simulink model "rfsoc4x2_ospfb_128"  (R2021a)
settings: Solver=VariableStepAuto  StartTime=0.0  StopTime=2048  RelTol=1e-3
undefined symbols (not defined in the file): pfb_coeff_gen_calc
libraries: xbsIndex_r4 x37092, casper_library_delays x737, casper_library_misc x68, xps_library x1
(part 128 of 339)

== system rfsoc4x2_ospfb_128/pfb_fir_real9/pol1_in1_tap27 ==
  din : Inport
  sync : Inport  Port=2
  coeff : Inport  Port=3
  addr_in : Inport  Port=4
  pot_en_in : Inport  Port=5
  Constant59 : xbsIndex_r4/Constant  const=0  gui_display_data_type=Fixed-point  arith_type=Unsigned  n_bits=16  bin_pt=0  preci_type=Single  exp_width=8  frac_width=24  explicit_period=off  period=1  equ=P=C  opselect=C  inp2=PCIN>>17  opr=+  inp1=P  carry=CIN  dbl_ovrd=off  block_type=constant
  Constant60 : xbsIndex_r4/Constant  const=0  gui_display_data_type=Boolean  arith_type=Boolean  n_bits=144  bin_pt=0  preci_type=Single  exp_width=8  frac_width=24  explicit_period=off  period=1  equ=P=C  opselect=C  inp2=PCIN>>17  opr=+  inp1=P  carry=CIN  dbl_ovrd=off  block_type=constant
  Delay : xbsIndex_r4/Delay  rst=off  infoeditControl=Selection of Reset will increase slice count due to use of real FFs and instead of SRLs  en=off  latency=1  reg_retiming=off  dbl_ovrd=off  block_type=delay
  Delay1 : xbsIndex_r4/Delay  rst=off  infoeditControl=Selection of Reset will increase slice count due to use of real FFs and instead of SRLs  en=off  latency=1  reg_retiming=off  dbl_ovrd=off  block_type=delay
  Dual Port RAM13 : xbsIndex_r4/Dual Port RAM  depth=(2^8) / (2^4)  initVector=0  distributed_mem=Block RAM  init_a=0  init_b=0  rst_a=off  rst_b=off  en_a=off  en_b=off  latency=1  write_mode_A=Read After Write  write_mode_B=Read Before Write  optimize=Area  dbl_ovrd=off  simulation_type=fast_sim  block_type=dpram
  Mult : xbsIndex_r4/Mult  precision=Full  arith_type="Signed  (2's comp)"  n_bits=8  bin_pt=2  quantization=Truncate  overflow=Wrap  en=off  latency=0  use_behavioral_HDL=on  opt=Speed  use_embedded=off  optimum_pipeline=off  pipeline=on  dbl_ovrd=off  use_rpm=on  placement_style=Rectangular shape  block_type=mult
      settings: xl_area=[0, 0, 0, 0, 0, 0, 0]  block_version=9.1.01
  Reinterpret : xbsIndex_r4/Reinterpret  force_arith_type=on  arith_type="Signed  (2's comp)"  force_bin_pt=on  bin_pt=coeff_frac_width  block_type=reinterpret
      settings: infoedit="Changes signal type without altering the binary representation.   You can changed the signal between signed and unsigned, and relocate the binary point.<P><P>Hardware notes: In hardware this block costs nothing.<P><P>Example:  Suppose the input is 6 bits wide, signed, with 2 fractional bits, and the output is forced to unsigned with 0 fractional bits.  Then an input of -2.0 (1110.00 in binary 2's complement) becomes an output of 56 (111000 in binary)."  block_version=9.1.01
  Reinterpret1 : xbsIndex_r4/Reinterpret  force_arith_type=on  arith_type="Signed  (2's comp)"  force_bin_pt=on  bin_pt=data_width - 1  block_type=reinterpret
      settings: infoedit="Changes signal type without altering the binary representation.   You can changed the signal between signed and unsigned, and relocate the binary point.<P><P>Hardware notes: In hardware this block costs nothing.<P><P>Example:  Suppose the input is 6 bits wide, signed, with 2 fractional bits, and the output is forced to unsigned with 0 fractional bits.  Then an input of -2.0 (1110.00 in binary 2's complement) becomes an output of 56 (111000 in binary)."  block_version=9.1.01
  Slice : xbsIndex_r4/Slice  nbits=coeff_width  boolean_output=off  mode=Lower Bit Location + Width  bit1=0  base1=MSB of Input  bit0=0  base0=LSB of Input  dbl_ovrd=off  block_type=slice
      settings: infoedit="Extracts a given range of bits from each input sample and presents it at the output.  The output type is ordinarily unsigned with binary point at zero, but can be Boolean when the slice is one bit wide.<P><P>Hardware notes: In hardware this block costs nothing."  block_version=9.1.01
  Slice1 : xbsIndex_r4/Slice  nbits=0  boolean_output=off  mode=Two Bit Locations  bit1=0  base1=MSB of Input  bit0=coeff_width  base0=LSB of Input  dbl_ovrd=off  block_type=slice
      settings: infoedit="Extracts a given range of bits from each input sample and presents it at the output.  The output type is ordinarily unsigned with binary point at zero, but can be Boolean when the slice is one bit wide.<P><P>Hardware notes: In hardware this block costs nothing."  block_version=9.1.01
  Terminator13 : Terminator
  delay_bram : Subsystem  Commented=on  AncestorBlock=casper_library_delays/delay_bram  mask(delay_bram){DelayLen=delay, bram_latency=bram_latency, use_dsp48=off, async=off}
      mask prompts: DelayLen "Delay By:"; bram_latency "BRAM Latency"; use_dsp48 "Use DSP48"; async "asynchronous operation"
      mask help: A delay block that uses BRAM for its storage.
      mask init:
      | delay_bram_init(gcb, ...
      |     'DelayLen', DelayLen, ...
      |     'bram_latency', bram_latency, ...
      |     'use_dsp48', use_dsp48, ...
      |     'async', async);
      mask Help: eval('xlWeb(''http://casper.berkeley.edu/wiki/Delay_bram'')')
  sync_delay : casper_library_delays/sync_delay  DelayLen=delay
      settings: SourceProductName=CASPER DSP Blockset
  dout : Outport  VectorParamsAs1DForOutWhenUnconnected=off
  sync_out : Outport  Port=2  VectorParamsAs1DForOutWhenUnconnected=off
  coeff_out : Outport  Port=3  VectorParamsAs1DForOutWhenUnconnected=off
  taps_out : Outport  Port=4  VectorParamsAs1DForOutWhenUnconnected=off
  add_out : Outport  Port=5  VectorParamsAs1DForOutWhenUnconnected=off
  pot_en_out : Outport  Port=6  VectorParamsAs1DForOutWhenUnconnected=off
  wires:
  addr_in/1 -> Dual Port RAM13/4, Dual Port RAM13/1, Delay/1
  pot_en_in/1 -> Delay1/1, Dual Port RAM13/3
  Constant59/1 -> Dual Port RAM13/5
  Constant60/1 -> Dual Port RAM13/6
  Dual Port RAM13/1 -> Terminator13/1
  din/1 -> Dual Port RAM13/2, Reinterpret1/1
  Delay/1 -> add_out/1
  Dual Port RAM13/2 -> dout/1
  Delay1/1 -> pot_en_out/1
  Reinterpret1/1 -> Mult/1
  Reinterpret/1 -> Mult/2
  Slice/1 -> Reinterpret/1
  Slice1/1 -> coeff_out/1
  coeff/1 -> Slice1/1, Slice/1
  sync_delay/1 -> sync_out/1
  sync/1 -> sync_delay/1
  Mult/1 -> taps_out/1

== system rfsoc4x2_ospfb_128/pfb_fir_real9/pol1_in1_tap28 ==
  note: 11 data in
  note: 12 data out
  din : Inport
  sync : Inport  Port=2
  coeff : Inport  Port=3
  addr_in : Inport  Port=4
  pot_en_in : Inport  Port=5
  Constant59 : xbsIndex_r4/Constant  const=0  gui_display_data_type=Fixed-point  arith_type=Unsigned  n_bits=16  bin_pt=0  preci_type=Single  exp_width=8  frac_width=24  explicit_period=off  period=1  equ=P=C  opselect=C  inp2=PCIN>>17  opr=+  inp1=P  carry=CIN  dbl_ovrd=off  block_type=constant
  Constant60 : xbsIndex_r4/Constant  const=0  gui_display_data_type=Boolean  arith_type=Boolean  n_bits=144  bin_pt=0  preci_type=Single  exp_width=8  frac_width=24  explicit_period=off  period=1  equ=P=C  opselect=C  inp2=PCIN>>17  opr=+  inp1=P  carry=CIN  dbl_ovrd=off  block_type=constant
  Dual Port RAM13 : xbsIndex_r4/Dual Port RAM  depth=(2^8) / (2^4)  initVector=0  distributed_mem=Block RAM  init_a=0  init_b=0  rst_a=off  rst_b=off  en_a=off  en_b=off  latency=1  write_mode_A=Read After Write  write_mode_B=Read Before Write  optimize=Area  dbl_ovrd=off  simulation_type=fast_sim  block_type=dpram
  Mult : xbsIndex_r4/Mult  precision=Full  arith_type="Signed  (2's comp)"  n_bits=8  bin_pt=2  quantization=Truncate  overflow=Wrap  en=off  latency=0  use_behavioral_HDL=on  opt=Speed  use_embedded=off  optimum_pipeline=off  pipeline=on  dbl_ovrd=off  use_rpm=on  placement_style=Rectangular shape  block_type=mult
      settings: xl_area=[0, 0, 0, 0, 0, 0, 0]  block_version=9.1.01
  Reinterpret : xbsIndex_r4/Reinterpret  force_arith_type=on  arith_type="Signed  (2's comp)"  force_bin_pt=on  bin_pt=coeff_frac_width  block_type=reinterpret
      settings: infoedit="Changes signal type without altering the binary representation.   You can changed the signal between signed and unsigned, and relocate the binary point.<P><P>Hardware notes: In hardware this block costs nothing.<P><P>Example:  Suppose the input is 6 bits wide, signed, with 2 fractional bits, and the output is forced to unsigned with 0 fractional bits.  Then an input of -2.0 (1110.00 in binary 2's complement) becomes an output of 56 (111000 in binary)."  block_version=9.1.01
  Reinterpret1 : xbsIndex_r4/Reinterpret  force_arith_type=on  arith_type="Signed  (2's comp)"  force_bin_pt=on  bin_pt=data_width - 1  block_type=reinterpret
      settings: infoedit="Changes signal type without altering the binary representation.   You can changed the signal between signed and unsigned, and relocate the binary point.<P><P>Hardware notes: In hardware this block costs nothing.<P><P>Example:  Suppose the input is 6 bits wide, signed, with 2 fractional bits, and the output is forced to unsigned with 0 fractional bits.  Then an input of -2.0 (1110.00 in binary 2's complement) becomes an output of 56 (111000 in binary)."  block_version=9.1.01
  Slice : xbsIndex_r4/Slice  nbits=coeff_width  boolean_output=off  mode=Lower Bit Location + Width  bit1=0  base1=MSB of Input  bit0=0  base0=LSB of Input  dbl_ovrd=off  block_type=slice
      settings: infoedit="Extracts a given range of bits from each input sample and presents it at the output.  The output type is ordinarily unsigned with binary point at zero, but can be Boolean when the slice is one bit wide.<P><P>Hardware notes: In hardware this block costs nothing."  block_version=9.1.01
  Slice1 : xbsIndex_r4/Slice  nbits=0  boolean_output=off  mode=Two Bit Locations  bit1=0  base1=MSB of Input  bit0=coeff_width  base0=LSB of Input  dbl_ovrd=off  block_type=slice
      settings: infoedit="Extracts a given range of bits from each input sample and presents it at the output.  The output type is ordinarily unsigned with binary point at zero, but can be Boolean when the slice is one bit wide.<P><P>Hardware notes: In hardware this block costs nothing."  block_version=9.1.01
  Terminator13 : Terminator
  delay_bram : Subsystem  Commented=on  AncestorBlock=casper_library_delays/delay_bram  mask(delay_bram){DelayLen=delay, bram_latency=bram_latency, use_dsp48=off, async=off}
      mask prompts: DelayLen "Delay By:"; bram_latency "BRAM Latency"; use_dsp48 "Use DSP48"; async "asynchronous operation"
      mask help: A delay block that uses BRAM for its storage.
      mask init:
      | delay_bram_init(gcb, ...
      |     'DelayLen', DelayLen, ...
      |     'bram_latency', bram_latency, ...
      |     'use_dsp48', use_dsp48, ...
      |     'async', async);
      mask Help: eval('xlWeb(''http://casper.berkeley.edu/wiki/Delay_bram'')')
  sync_delay : casper_library_delays/sync_delay  DelayLen=delay
      settings: SourceProductName=CASPER DSP Blockset
  dout : Outport  VectorParamsAs1DForOutWhenUnconnected=off
  sync_out : Outport  Port=2  VectorParamsAs1DForOutWhenUnconnected=off
  coeff_out : Outport  Port=3  VectorParamsAs1DForOutWhenUnconnected=off
  taps_out : Outport  Port=4  VectorParamsAs1DForOutWhenUnconnected=off
  wires:
  Dual Port RAM13/1 -> Terminator13/1
  Dual Port RAM13/2 -> dout/1
  Constant59/1 -> Dual Port RAM13/5
  Constant60/1 -> Dual Port RAM13/6
  din/1 -> Dual Port RAM13/2, Reinterpret1/1
  addr_in/1 -> Dual Port RAM13/1, Dual Port RAM13/4
  pot_en_in/1 -> Dual Port RAM13/3
  Reinterpret1/1 -> Mult/1
  Reinterpret/1 -> Mult/2
  Slice/1 -> Reinterpret/1
  Slice1/1 -> coeff_out/1
  coeff/1 -> Slice1/1, Slice/1
  sync_delay/1 -> sync_out/1
  sync/1 -> sync_delay/1
  Mult/1 -> taps_out/1

== system rfsoc4x2_ospfb_128/pfb_fir_real9/pol1_in1_tap29 ==
  din : Inport
  sync : Inport  Port=2
  coeff : Inport  Port=3
  addr_in : Inport  Port=4
  pot_en_in : Inport  Port=5
  Constant59 : xbsIndex_r4/Constant  const=0  gui_display_data_type=Fixed-point  arith_type=Unsigned  n_bits=16  bin_pt=0  preci_type=Single  exp_width=8  frac_width=24  explicit_period=off  period=1  equ=P=C  opselect=C  inp2=PCIN>>17  opr=+  inp1=P  carry=CIN  dbl_ovrd=off  block_type=constant
  Constant60 : xbsIndex_r4/Constant  const=0  gui_display_data_type=Boolean  arith_type=Boolean  n_bits=144  bin_pt=0  preci_type=Single  exp_width=8  frac_width=24  explicit_period=off  period=1  equ=P=C  opselect=C  inp2=PCIN>>17  opr=+  inp1=P  carry=CIN  dbl_ovrd=off  block_type=constant
  Delay : xbsIndex_r4/Delay  rst=off  infoeditControl=Selection of Reset will increase slice count due to use of real FFs and instead of SRLs  en=off  latency=1  reg_retiming=off  dbl_ovrd=off  block_type=delay
  Delay1 : xbsIndex_r4/Delay  rst=off  infoeditControl=Selection of Reset will increase slice count due to use of real FFs and instead of SRLs  en=off  latency=1  reg_retiming=off  dbl_ovrd=off  block_type=delay
  Dual Port RAM13 : xbsIndex_r4/Dual Port RAM  depth=(2^8) / (2^4)  initVector=0  distributed_mem=Block RAM  init_a=0  init_b=0  rst_a=off  rst_b=off  en_a=off  en_b=off  latency=1  write_mode_A=Read After Write  write_mode_B=Read Before Write  optimize=Area  dbl_ovrd=off  simulation_type=fast_sim  block_type=dpram
  Mult : xbsIndex_r4/Mult  precision=Full  arith_type="Signed  (2's comp)"  n_bits=8  bin_pt=2  quantization=Truncate  overflow=Wrap  en=off  latency=0  use_behavioral_HDL=on  opt=Speed  use_embedded=off  optimum_pipeline=off  pipeline=on  dbl_ovrd=off  use_rpm=on  placement_style=Rectangular shape  block_type=mult
      settings: xl_area=[0, 0, 0, 0, 0, 0, 0]  block_version=9.1.01
  Reinterpret : xbsIndex_r4/Reinterpret  force_arith_type=on  arith_type="Signed  (2's comp)"  force_bin_pt=on  bin_pt=coeff_frac_width  block_type=reinterpret
      settings: infoedit="Changes signal type without altering the binary representation.   You can changed the signal between signed and unsigned, and relocate the binary point.<P><P>Hardware notes: In hardware this block costs nothing.<P><P>Example:  Suppose the input is 6 bits wide, signed, with 2 fractional bits, and the output is forced to unsigned with 0 fractional bits.  Then an input of -2.0 (1110.00 in binary 2's complement) becomes an output of 56 (111000 in binary)."  block_version=9.1.01
  Reinterpret1 : xbsIndex_r4/Reinterpret  force_arith_type=on  arith_type="Signed  (2's comp)"  force_bin_pt=on  bin_pt=data_width - 1  block_type=reinterpret
      settings: infoedit="Changes signal type without altering the binary representation.   You can changed the signal between signed and unsigned, and relocate the binary point.<P><P>Hardware notes: In hardware this block costs nothing.<P><P>Example:  Suppose the input is 6 bits wide, signed, with 2 fractional bits, and the output is forced to unsigned with 0 fractional bits.  Then an input of -2.0 (1110.00 in binary 2's complement) becomes an output of 56 (111000 in binary)."  block_version=9.1.01
  Slice : xbsIndex_r4/Slice  nbits=coeff_width  boolean_output=off  mode=Lower Bit Location + Width  bit1=0  base1=MSB of Input  bit0=0  base0=LSB of Input  dbl_ovrd=off  block_type=slice
      settings: infoedit="Extracts a given range of bits from each input sample and presents it at the output.  The output type is ordinarily unsigned with binary point at zero, but can be Boolean when the slice is one bit wide.<P><P>Hardware notes: In hardware this block costs nothing."  block_version=9.1.01
  Slice1 : xbsIndex_r4/Slice  nbits=0  boolean_output=off  mode=Two Bit Locations  bit1=0  base1=MSB of Input  bit0=coeff_width  base0=LSB of Input  dbl_ovrd=off  block_type=slice
      settings: infoedit="Extracts a given range of bits from each input sample and presents it at the output.  The output type is ordinarily unsigned with binary point at zero, but can be Boolean when the slice is one bit wide.<P><P>Hardware notes: In hardware this block costs nothing."  block_version=9.1.01
  Terminator13 : Terminator
  delay_bram : Subsystem  Commented=on  AncestorBlock=casper_library_delays/delay_bram  mask(delay_bram){DelayLen=delay, bram_latency=bram_latency, use_dsp48=off, async=off}
      mask prompts: DelayLen "Delay By:"; bram_latency "BRAM Latency"; use_dsp48 "Use DSP48"; async "asynchronous operation"
      mask help: A delay block that uses BRAM for its storage.
      mask init:
      | delay_bram_init(gcb, ...
      |     'DelayLen', DelayLen, ...
      |     'bram_latency', bram_latency, ...
      |     'use_dsp48', use_dsp48, ...
      |     'async', async);
      mask Help: eval('xlWeb(''http://casper.berkeley.edu/wiki/Delay_bram'')')
  sync_delay : casper_library_delays/sync_delay  DelayLen=delay
      settings: SourceProductName=CASPER DSP Blockset
  dout : Outport  VectorParamsAs1DForOutWhenUnconnected=off
  sync_out : Outport  Port=2  VectorParamsAs1DForOutWhenUnconnected=off
  coeff_out : Outport  Port=3  VectorParamsAs1DForOutWhenUnconnected=off
  taps_out : Outport  Port=4  VectorParamsAs1DForOutWhenUnconnected=off
  add_out : Outport  Port=5  VectorParamsAs1DForOutWhenUnconnected=off
  pot_en_out : Outport  Port=6  VectorParamsAs1DForOutWhenUnconnected=off
  wires:
  pot_en_in/1 -> Delay1/1, Dual Port RAM13/3
  Constant59/1 -> Dual Port RAM13/5
  Dual Port RAM13/1 -> Terminator13/1
  Dual Port RAM13/2 -> dout/1
  addr_in/1 -> Dual Port RAM13/4, Dual Port RAM13/1, Delay/1
  Delay/1 -> add_out/1
  Delay1/1 -> pot_en_out/1
  din/1 -> Dual Port RAM13/2, Reinterpret1/1
  Constant60/1 -> Dual Port RAM13/6
  Reinterpret1/1 -> Mult/1
  Reinterpret/1 -> Mult/2
  Slice/1 -> Reinterpret/1
  Slice1/1 -> coeff_out/1
  coeff/1 -> Slice1/1, Slice/1
  sync_delay/1 -> sync_out/1
  sync/1 -> sync_delay/1
  Mult/1 -> taps_out/1

== system rfsoc4x2_ospfb_128/pfb_fir_real9/pol1_in1_tap3 ==
  din : Inport
  sync : Inport  Port=2
  coeff : Inport  Port=3
  addr_in : Inport  Port=4
  pot_en_in : Inport  Port=5
  Constant59 : xbsIndex_r4/Constant  const=0  gui_display_data_type=Fixed-point  arith_type=Unsigned  n_bits=16  bin_pt=0  preci_type=Single  exp_width=8  frac_width=24  explicit_period=off  period=1  equ=P=C  opselect=C  inp2=PCIN>>17  opr=+  inp1=P  carry=CIN  dbl_ovrd=off  block_type=constant
  Constant60 : xbsIndex_r4/Constant  const=0  gui_display_data_type=Boolean  arith_type=Boolean  n_bits=144  bin_pt=0  preci_type=Single  exp_width=8  frac_width=24  explicit_period=off  period=1  equ=P=C  opselect=C  inp2=PCIN>>17  opr=+  inp1=P  carry=CIN  dbl_ovrd=off  block_type=constant
  Delay : xbsIndex_r4/Delay  rst=off  infoeditControl=Selection of Reset will increase slice count due to use of real FFs and instead of SRLs  en=off  latency=1  reg_retiming=off  dbl_ovrd=off  block_type=delay
  Delay1 : xbsIndex_r4/Delay  rst=off  infoeditControl=Selection of Reset will increase slice count due to use of real FFs and instead of SRLs  en=off  latency=1  reg_retiming=off  dbl_ovrd=off  block_type=delay
  Dual Port RAM13 : xbsIndex_r4/Dual Port RAM  depth=(2^8) / (2^4)  initVector=0  distributed_mem=Block RAM  init_a=0  init_b=0  rst_a=off  rst_b=off  en_a=off  en_b=off  latency=1  write_mode_A=Read After Write  write_mode_B=Read Before Write  optimize=Area  dbl_ovrd=off  simulation_type=fast_sim  block_type=dpram
  Mult : xbsIndex_r4/Mult  precision=Full  arith_type="Signed  (2's comp)"  n_bits=8  bin_pt=2  quantization=Truncate  overflow=Wrap  en=off  latency=0  use_behavioral_HDL=on  opt=Speed  use_embedded=off  optimum_pipeline=off  pipeline=on  dbl_ovrd=off  use_rpm=on  placement_style=Rectangular shape  block_type=mult
      settings: xl_area=[0, 0, 0, 0, 0, 0, 0]  block_version=9.1.01
  Reinterpret : xbsIndex_r4/Reinterpret  force_arith_type=on  arith_type="Signed  (2's comp)"  force_bin_pt=on  bin_pt=coeff_frac_width  block_type=reinterpret
      settings: infoedit="Changes signal type without altering the binary representation.   You can changed the signal between signed and unsigned, and relocate the binary point.<P><P>Hardware notes: In hardware this block costs nothing.<P><P>Example:  Suppose the input is 6 bits wide, signed, with 2 fractional bits, and the output is forced to unsigned with 0 fractional bits.  Then an input of -2.0 (1110.00 in binary 2's complement) becomes an output of 56 (111000 in binary)."  block_version=9.1.01
  Reinterpret1 : xbsIndex_r4/Reinterpret  force_arith_type=on  arith_type="Signed  (2's comp)"  force_bin_pt=on  bin_pt=data_width - 1  block_type=reinterpret
      settings: infoedit="Changes signal type without altering the binary representation.   You can changed the signal between signed and unsigned, and relocate the binary point.<P><P>Hardware notes: In hardware this block costs nothing.<P><P>Example:  Suppose the input is 6 bits wide, signed, with 2 fractional bits, and the output is forced to unsigned with 0 fractional bits.  Then an input of -2.0 (1110.00 in binary 2's complement) becomes an output of 56 (111000 in binary)."  block_version=9.1.01
  Slice : xbsIndex_r4/Slice  nbits=coeff_width  boolean_output=off  mode=Lower Bit Location + Width  bit1=0  base1=MSB of Input  bit0=0  base0=LSB of Input  dbl_ovrd=off  block_type=slice
      settings: infoedit="Extracts a given range of bits from each input sample and presents it at the output.  The output type is ordinarily unsigned with binary point at zero, but can be Boolean when the slice is one bit wide.<P><P>Hardware notes: In hardware this block costs nothing."  block_version=9.1.01
  Slice1 : xbsIndex_r4/Slice  nbits=0  boolean_output=off  mode=Two Bit Locations  bit1=0  base1=MSB of Input  bit0=coeff_width  base0=LSB of Input  dbl_ovrd=off  block_type=slice
      settings: infoedit="Extracts a given range of bits from each input sample and presents it at the output.  The output type is ordinarily unsigned with binary point at zero, but can be Boolean when the slice is one bit wide.<P><P>Hardware notes: In hardware this block costs nothing."  block_version=9.1.01
  Terminator13 : Terminator
  delay_bram : Subsystem  Commented=on  AncestorBlock=casper_library_delays/delay_bram  mask(delay_bram){DelayLen=delay, bram_latency=bram_latency, use_dsp48=off, async=off}
      mask prompts: DelayLen "Delay By:"; bram_latency "BRAM Latency"; use_dsp48 "Use DSP48"; async "asynchronous operation"
      mask help: A delay block that uses BRAM for its storage.
      mask init:
      | delay_bram_init(gcb, ...
      |     'DelayLen', DelayLen, ...
      |     'bram_latency', bram_latency, ...
      |     'use_dsp48', use_dsp48, ...
      |     'async', async);
      mask Help: eval('xlWeb(''http://casper.berkeley.edu/wiki/Delay_bram'')')
  sync_delay : casper_library_delays/sync_delay  DelayLen=delay
      settings: SourceProductName=CASPER DSP Blockset
  dout : Outport  VectorParamsAs1DForOutWhenUnconnected=off
  sync_out : Outport  Port=2  VectorParamsAs1DForOutWhenUnconnected=off
  coeff_out : Outport  Port=3  VectorParamsAs1DForOutWhenUnconnected=off
  taps_out : Outport  Port=4  VectorParamsAs1DForOutWhenUnconnected=off
  add_out : Outport  Port=5  VectorParamsAs1DForOutWhenUnconnected=off
  pot_en_out : Outport  Port=6  VectorParamsAs1DForOutWhenUnconnected=off
  wires:
  Mult/1 -> taps_out/1
  sync/1 -> sync_delay/1
  sync_delay/1 -> sync_out/1
  coeff/1 -> Slice/1, Slice1/1
  Slice1/1 -> coeff_out/1
  Slice/1 -> Reinterpret/1
  Reinterpret/1 -> Mult/2
  Reinterpret1/1 -> Mult/1
  Constant60/1 -> Dual Port RAM13/6
  din/1 -> Reinterpret1/1, Dual Port RAM13/2
  Delay1/1 -> pot_en_out/1
  Delay/1 -> add_out/1
  addr_in/1 -> Delay/1, Dual Port RAM13/1, Dual Port RAM13/4
  Dual Port RAM13/2 -> dout/1
  Dual Port RAM13/1 -> Terminator13/1
  Constant59/1 -> Dual Port RAM13/5
  pot_en_in/1 -> Dual Port RAM13/3, Delay1/1

== system rfsoc4x2_ospfb_128/pfb_fir_real9/pol1_in1_tap30 ==
  din : Inport
  sync : Inport  Port=2
  coeff : Inport  Port=3
  addr_in : Inport  Port=4
  pot_en_in : Inport  Port=5
  Constant59 : xbsIndex_r4/Constant  const=0  gui_display_data_type=Fixed-point  arith_type=Unsigned  n_bits=16  bin_pt=0  preci_type=Single  exp_width=8  frac_width=24  explicit_period=off  period=1  equ=P=C  opselect=C  inp2=PCIN>>17  opr=+  inp1=P  carry=CIN  dbl_ovrd=off  block_type=constant
  Constant60 : xbsIndex_r4/Constant  const=0  gui_display_data_type=Boolean  arith_type=Boolean  n_bits=144  bin_pt=0  preci_type=Single  exp_width=8  frac_width=24  explicit_period=off  period=1  equ=P=C  opselect=C  inp2=PCIN>>17  opr=+  inp1=P  carry=CIN  dbl_ovrd=off  block_type=constant
  Delay : xbsIndex_r4/Delay  rst=off  infoeditControl=Selection of Reset will increase slice count due to use of real FFs and instead of SRLs  en=off  latency=1  reg_retiming=off  dbl_ovrd=off  block_type=delay
  Delay1 : xbsIndex_r4/Delay  rst=off  infoeditControl=Selection of Reset will increase slice count due to use of real FFs and instead of SRLs  en=off  latency=1  reg_retiming=off  dbl_ovrd=off  block_type=delay
  Dual Port RAM13 : xbsIndex_r4/Dual Port RAM  depth=(2^8) / (2^4)  initVector=0  distributed_mem=Block RAM  init_a=0  init_b=0  rst_a=off  rst_b=off  en_a=off  en_b=off  latency=1  write_mode_A=Read After Write  write_mode_B=Read Before Write  optimize=Area  dbl_ovrd=off  simulation_type=fast_sim  block_type=dpram
  Mult : xbsIndex_r4/Mult  precision=Full  arith_type="Signed  (2's comp)"  n_bits=8  bin_pt=2  quantization=Truncate  overflow=Wrap  en=off  latency=0  use_behavioral_HDL=on  opt=Speed  use_embedded=off  optimum_pipeline=off  pipeline=on  dbl_ovrd=off  use_rpm=on  placement_style=Rectangular shape  block_type=mult
      settings: xl_area=[0, 0, 0, 0, 0, 0, 0]  block_version=9.1.01
  Reinterpret : xbsIndex_r4/Reinterpret  force_arith_type=on  arith_type="Signed  (2's comp)"  force_bin_pt=on  bin_pt=coeff_frac_width  block_type=reinterpret
      settings: infoedit="Changes signal type without altering the binary representation.   You can changed the signal between signed and unsigned, and relocate the binary point.<P><P>Hardware notes: In hardware this block costs nothing.<P><P>Example:  Suppose the input is 6 bits wide, signed, with 2 fractional bits, and the output is forced to unsigned with 0 fractional bits.  Then an input of -2.0 (1110.00 in binary 2's complement) becomes an output of 56 (111000 in binary)."  block_version=9.1.01
  Reinterpret1 : xbsIndex_r4/Reinterpret  force_arith_type=on  arith_type="Signed  (2's comp)"  force_bin_pt=on  bin_pt=data_width - 1  block_type=reinterpret
      settings: infoedit="Changes signal type without altering the binary representation.   You can changed the signal between signed and unsigned, and relocate the binary point.<P><P>Hardware notes: In hardware this block costs nothing.<P><P>Example:  Suppose the input is 6 bits wide, signed, with 2 fractional bits, and the output is forced to unsigned with 0 fractional bits.  Then an input of -2.0 (1110.00 in binary 2's complement) becomes an output of 56 (111000 in binary)."  block_version=9.1.01
  Slice : xbsIndex_r4/Slice  nbits=coeff_width  boolean_output=off  mode=Lower Bit Location + Width  bit1=0  base1=MSB of Input  bit0=0  base0=LSB of Input  dbl_ovrd=off  block_type=slice
      settings: infoedit="Extracts a given range of bits from each input sample and presents it at the output.  The output type is ordinarily unsigned with binary point at zero, but can be Boolean when the slice is one bit wide.<P><P>Hardware notes: In hardware this block costs nothing."  block_version=9.1.01
  Slice1 : xbsIndex_r4/Slice  nbits=0  boolean_output=off  mode=Two Bit Locations  bit1=0  base1=MSB of Input  bit0=coeff_width  base0=LSB of Input  dbl_ovrd=off  block_type=slice
      settings: infoedit="Extracts a given range of bits from each input sample and presents it at the output.  The output type is ordinarily unsigned with binary point at zero, but can be Boolean when the slice is one bit wide.<P><P>Hardware notes: In hardware this block costs nothing."  block_version=9.1.01
  Terminator13 : Terminator
  delay_bram : Subsystem  Commented=on  AncestorBlock=casper_library_delays/delay_bram  mask(delay_bram){DelayLen=delay, bram_latency=bram_latency, use_dsp48=off, async=off}
      mask prompts: DelayLen "Delay By:"; bram_latency "BRAM Latency"; use_dsp48 "Use DSP48"; async "asynchronous operation"
      mask help: A delay block that uses BRAM for its storage.
      mask init:
      | delay_bram_init(gcb, ...
      |     'DelayLen', DelayLen, ...
      |     'bram_latency', bram_latency, ...
      |     'use_dsp48', use_dsp48, ...
      |     'async', async);
      mask Help: eval('xlWeb(''http://casper.berkeley.edu/wiki/Delay_bram'')')
  sync_delay : casper_library_delays/sync_delay  DelayLen=delay
      settings: SourceProductName=CASPER DSP Blockset
  dout : Outport  VectorParamsAs1DForOutWhenUnconnected=off
  sync_out : Outport  Port=2  VectorParamsAs1DForOutWhenUnconnected=off
  coeff_out : Outport  Port=3  VectorParamsAs1DForOutWhenUnconnected=off
  taps_out : Outport  Port=4  VectorParamsAs1DForOutWhenUnconnected=off
  add_out : Outport  Port=5  VectorParamsAs1DForOutWhenUnconnected=off
  pot_en_out : Outport  Port=6  VectorParamsAs1DForOutWhenUnconnected=off
  wires:
  addr_in/1 -> Dual Port RAM13/4, Dual Port RAM13/1, Delay/1
  pot_en_in/1 -> Delay1/1, Dual Port RAM13/3
  Constant59/1 -> Dual Port RAM13/5
  Constant60/1 -> Dual Port RAM13/6
  Dual Port RAM13/1 -> Terminator13/1
  din/1 -> Reinterpret1/1, Dual Port RAM13/2
  Delay/1 -> add_out/1
  Dual Port RAM13/2 -> dout/1
  Delay1/1 -> pot_en_out/1
  Reinterpret1/1 -> Mult/1
  Reinterpret/1 -> Mult/2
  Slice/1 -> Reinterpret/1
  Slice1/1 -> coeff_out/1
  coeff/1 -> Slice1/1, Slice/1
  sync_delay/1 -> sync_out/1
  sync/1 -> sync_delay/1
  Mult/1 -> taps_out/1

== system rfsoc4x2_ospfb_128/pfb_fir_real9/pol1_in1_tap31 ==
  note: 10 data in
  note: 11 data out
  din : Inport
  sync : Inport  Port=2
  coeff : Inport  Port=3
  addr_in : Inport  Port=4
  pot_en_in : Inport  Port=5
  Constant59 : xbsIndex_r4/Constant  const=0  gui_display_data_type=Fixed-point  arith_type=Unsigned  n_bits=16  bin_pt=0  preci_type=Single  exp_width=8  frac_width=24  explicit_period=off  period=1  equ=P=C  opselect=C  inp2=PCIN>>17  opr=+  inp1=P  carry=CIN  dbl_ovrd=off  block_type=constant
  Constant60 : xbsIndex_r4/Constant  const=0  gui_display_data_type=Boolean  arith_type=Boolean  n_bits=144  bin_pt=0  preci_type=Single  exp_width=8  frac_width=24  explicit_period=off  period=1  equ=P=C  opselect=C  inp2=PCIN>>17  opr=+  inp1=P  carry=CIN  dbl_ovrd=off  block_type=constant
  Delay : xbsIndex_r4/Delay  rst=off  infoeditControl=Selection of Reset will increase slice count due to use of real FFs and instead of SRLs  en=off  latency=1  reg_retiming=off  dbl_ovrd=off  block_type=delay
  Delay1 : xbsIndex_r4/Delay  rst=off  infoeditControl=Selection of Reset will increase slice count due to use of real FFs and instead of SRLs  en=off  latency=1  reg_retiming=off  dbl_ovrd=off  block_type=delay
  Dual Port RAM13 : xbsIndex_r4/Dual Port RAM  depth=(2^8) / (2^4)  initVector=0  distributed_mem=Block RAM  init_a=0  init_b=0  rst_a=off  rst_b=off  en_a=off  en_b=off  latency=1  write_mode_A=Read After Write  write_mode_B=Read Before Write  optimize=Area  dbl_ovrd=off  simulation_type=fast_sim  block_type=dpram
  Mult : xbsIndex_r4/Mult  precision=Full  arith_type="Signed  (2's comp)"  n_bits=8  bin_pt=2  quantization=Truncate  overflow=Wrap  en=off  latency=0  use_behavioral_HDL=on  opt=Speed  use_embedded=off  optimum_pipeline=off  pipeline=on  dbl_ovrd=off  use_rpm=on  placement_style=Rectangular shape  block_type=mult
      settings: xl_area=[0, 0, 0, 0, 0, 0, 0]  block_version=9.1.01
  Reinterpret : xbsIndex_r4/Reinterpret  force_arith_type=on  arith_type="Signed  (2's comp)"  force_bin_pt=on  bin_pt=coeff_frac_width  block_type=reinterpret
      settings: infoedit="Changes signal type without altering the binary representation.   You can changed the signal between signed and unsigned, and relocate the binary point.<P><P>Hardware notes: In hardware this block costs nothing.<P><P>Example:  Suppose the input is 6 bits wide, signed, with 2 fractional bits, and the output is forced to unsigned with 0 fractional bits.  Then an input of -2.0 (1110.00 in binary 2's complement) becomes an output of 56 (111000 in binary)."  block_version=9.1.01
  Reinterpret1 : xbsIndex_r4/Reinterpret  force_arith_type=on  arith_type="Signed  (2's comp)"  force_bin_pt=on  bin_pt=data_width - 1  block_type=reinterpret
      settings: infoedit="Changes signal type without altering the binary representation.   You can changed the signal between signed and unsigned, and relocate the binary point.<P><P>Hardware notes: In hardware this block costs nothing.<P><P>Example:  Suppose the input is 6 bits wide, signed, with 2 fractional bits, and the output is forced to unsigned with 0 fractional bits.  Then an input of -2.0 (1110.00 in binary 2's complement) becomes an output of 56 (111000 in binary)."  block_version=9.1.01
  Slice : xbsIndex_r4/Slice  nbits=coeff_width  boolean_output=off  mode=Lower Bit Location + Width  bit1=0  base1=MSB of Input  bit0=0  base0=LSB of Input  dbl_ovrd=off  block_type=slice
      settings: infoedit="Extracts a given range of bits from each input sample and presents it at the output.  The output type is ordinarily unsigned with binary point at zero, but can be Boolean when the slice is one bit wide.<P><P>Hardware notes: In hardware this block costs nothing."  block_version=9.1.01
  Slice1 : xbsIndex_r4/Slice  nbits=0  boolean_output=off  mode=Two Bit Locations  bit1=0  base1=MSB of Input  bit0=coeff_width  base0=LSB of Input  dbl_ovrd=off  block_type=slice
      settings: infoedit="Extracts a given range of bits from each input sample and presents it at the output.  The output type is ordinarily unsigned with binary point at zero, but can be Boolean when the slice is one bit wide.<P><P>Hardware notes: In hardware this block costs nothing."  block_version=9.1.01
  Terminator13 : Terminator
  delay_bram : Subsystem  Commented=on  AncestorBlock=casper_library_delays/delay_bram  mask(delay_bram){DelayLen=delay, bram_latency=bram_latency, use_dsp48=off, async=off}
      mask prompts: DelayLen "Delay By:"; bram_latency "BRAM Latency"; use_dsp48 "Use DSP48"; async "asynchronous operation"
      mask help: A delay block that uses BRAM for its storage.
      mask init:
      | delay_bram_init(gcb, ...
      |     'DelayLen', DelayLen, ...
      |     'bram_latency', bram_latency, ...
      |     'use_dsp48', use_dsp48, ...
      |     'async', async);
      mask Help: eval('xlWeb(''http://casper.berkeley.edu/wiki/Delay_bram'')')
  sync_delay : casper_library_delays/sync_delay  DelayLen=delay
      settings: SourceProductName=CASPER DSP Blockset
  dout : Outport  VectorParamsAs1DForOutWhenUnconnected=off
  sync_out : Outport  Port=2  VectorParamsAs1DForOutWhenUnconnected=off
  coeff_out : Outport  Port=3  VectorParamsAs1DForOutWhenUnconnected=off
  taps_out : Outport  Port=4  VectorParamsAs1DForOutWhenUnconnected=off
  add_out : Outport  Port=5  VectorParamsAs1DForOutWhenUnconnected=off
  pot_en_out : Outport  Port=6  VectorParamsAs1DForOutWhenUnconnected=off
  wires:
  Constant60/1 -> Dual Port RAM13/6
  Delay1/1 -> pot_en_out/1
  Dual Port RAM13/1 -> Terminator13/1
  pot_en_in/1 -> Delay1/1, Dual Port RAM13/3
  Constant59/1 -> Dual Port RAM13/5
  addr_in/1 -> Dual Port RAM13/4, Dual Port RAM13/1, Delay/1
  Dual Port RAM13/2 -> dout/1
  Delay/1 -> add_out/1
  din/1 -> Dual Port RAM13/2, Reinterpret1/1
  Reinterpret1/1 -> Mult/1
  Reinterpret/1 -> Mult/2
  Slice/1 -> Reinterpret/1
  Slice1/1 -> coeff_out/1
  coeff/1 -> Slice1/1, Slice/1
  sync_delay/1 -> sync_out/1
  sync/1 -> sync_delay/1
  Mult/1 -> taps_out/1

== system rfsoc4x2_ospfb_128/pfb_fir_real9/pol1_in1_tap32 ==
  din : Inport
  sync : Inport  Port=2
  coeff : Inport  Port=3
  addr_in : Inport  Port=4
  pot_en_in : Inport  Port=5
  Constant59 : xbsIndex_r4/Constant  const=0  gui_display_data_type=Fixed-point  arith_type=Unsigned  n_bits=16  bin_pt=0  preci_type=Single  exp_width=8  frac_width=24  explicit_period=off  period=1  equ=P=C  opselect=C  inp2=PCIN>>17  opr=+  inp1=P  carry=CIN  dbl_ovrd=off  block_type=constant
  Constant60 : xbsIndex_r4/Constant  const=0  gui_display_data_type=Boolean  arith_type=Boolean  n_bits=144  bin_pt=0  preci_type=Single  exp_width=8  frac_width=24  explicit_period=off  period=1  equ=P=C  opselect=C  inp2=PCIN>>17  opr=+  inp1=P  carry=CIN  dbl_ovrd=off  block_type=constant
  Delay : xbsIndex_r4/Delay  rst=off  infoeditControl=Selection of Reset will increase slice count due to use of real FFs and instead of SRLs  en=off  latency=1  reg_retiming=off  dbl_ovrd=off  block_type=delay
  Delay1 : xbsIndex_r4/Delay  rst=off  infoeditControl=Selection of Reset will increase slice count due to use of real FFs and instead of SRLs  en=off  latency=1  reg_retiming=off  dbl_ovrd=off  block_type=delay
  Dual Port RAM13 : xbsIndex_r4/Dual Port RAM  depth=(2^8) / (2^4)  initVector=0  distributed_mem=Block RAM  init_a=0  init_b=0  rst_a=off  rst_b=off  en_a=off  en_b=off  latency=1  write_mode_A=Read After Write  write_mode_B=Read Before Write  optimize=Area  dbl_ovrd=off  simulation_type=fast_sim  block_type=dpram
  Mult : xbsIndex_r4/Mult  precision=Full  arith_type="Signed  (2's comp)"  n_bits=8  bin_pt=2  quantization=Truncate  overflow=Wrap  en=off  latency=0  use_behavioral_HDL=on  opt=Speed  use_embedded=off  optimum_pipeline=off  pipeline=on  dbl_ovrd=off  use_rpm=on  placement_style=Rectangular shape  block_type=mult
      settings: xl_area=[0, 0, 0, 0, 0, 0, 0]  block_version=9.1.01
  Reinterpret : xbsIndex_r4/Reinterpret  force_arith_type=on  arith_type="Signed  (2's comp)"  force_bin_pt=on  bin_pt=coeff_frac_width  block_type=reinterpret
      settings: infoedit="Changes signal type without altering the binary representation.   You can changed the signal between signed and unsigned, and relocate the binary point.<P><P>Hardware notes: In hardware this block costs nothing.<P><P>Example:  Suppose the input is 6 bits wide, signed, with 2 fractional bits, and the output is forced to unsigned with 0 fractional bits.  Then an input of -2.0 (1110.00 in binary 2's complement) becomes an output of 56 (111000 in binary)."  block_version=9.1.01
  Reinterpret1 : xbsIndex_r4/Reinterpret  force_arith_type=on  arith_type="Signed  (2's comp)"  force_bin_pt=on  bin_pt=data_width - 1  block_type=reinterpret
      settings: infoedit="Changes signal type without altering the binary representation.   You can changed the signal between signed and unsigned, and relocate the binary point.<P><P>Hardware notes: In hardware this block costs nothing.<P><P>Example:  Suppose the input is 6 bits wide, signed, with 2 fractional bits, and the output is forced to unsigned with 0 fractional bits.  Then an input of -2.0 (1110.00 in binary 2's complement) becomes an output of 56 (111000 in binary)."  block_version=9.1.01
  Slice : xbsIndex_r4/Slice  nbits=coeff_width  boolean_output=off  mode=Lower Bit Location + Width  bit1=0  base1=MSB of Input  bit0=0  base0=LSB of Input  dbl_ovrd=off  block_type=slice
      settings: infoedit="Extracts a given range of bits from each input sample and presents it at the output.  The output type is ordinarily unsigned with binary point at zero, but can be Boolean when the slice is one bit wide.<P><P>Hardware notes: In hardware this block costs nothing."  block_version=9.1.01
  Slice1 : xbsIndex_r4/Slice  nbits=0  boolean_output=off  mode=Two Bit Locations  bit1=0  base1=MSB of Input  bit0=coeff_width  base0=LSB of Input  dbl_ovrd=off  block_type=slice
      settings: infoedit="Extracts a given range of bits from each input sample and presents it at the output.  The output type is ordinarily unsigned with binary point at zero, but can be Boolean when the slice is one bit wide.<P><P>Hardware notes: In hardware this block costs nothing."  block_version=9.1.01
  Terminator13 : Terminator
  delay_bram : Subsystem  Commented=on  AncestorBlock=casper_library_delays/delay_bram  mask(delay_bram){DelayLen=delay, bram_latency=bram_latency, use_dsp48=off, async=off}
      mask prompts: DelayLen "Delay By:"; bram_latency "BRAM Latency"; use_dsp48 "Use DSP48"; async "asynchronous operation"
      mask help: A delay block that uses BRAM for its storage.
      mask init:
      | delay_bram_init(gcb, ...
      |     'DelayLen', DelayLen, ...
      |     'bram_latency', bram_latency, ...
      |     'use_dsp48', use_dsp48, ...
      |     'async', async);
      mask Help: eval('xlWeb(''http://casper.berkeley.edu/wiki/Delay_bram'')')
  sync_delay : casper_library_delays/sync_delay  DelayLen=delay
      settings: SourceProductName=CASPER DSP Blockset
  dout : Outport  VectorParamsAs1DForOutWhenUnconnected=off
  sync_out : Outport  Port=2  VectorParamsAs1DForOutWhenUnconnected=off
  coeff_out : Outport  Port=3  VectorParamsAs1DForOutWhenUnconnected=off
  taps_out : Outport  Port=4  VectorParamsAs1DForOutWhenUnconnected=off
  add_out : Outport  Port=5  VectorParamsAs1DForOutWhenUnconnected=off
  pot_en_out : Outport  Port=6  VectorParamsAs1DForOutWhenUnconnected=off
  wires:
  addr_in/1 -> Dual Port RAM13/4, Dual Port RAM13/1, Delay/1
  pot_en_in/1 -> Delay1/1, Dual Port RAM13/3
  Constant59/1 -> Dual Port RAM13/5
  Constant60/1 -> Dual Port RAM13/6
  Dual Port RAM13/1 -> Terminator13/1
  din/1 -> Reinterpret1/1, Dual Port RAM13/2
  Delay/1 -> add_out/1
  Dual Port RAM13/2 -> dout/1
  Delay1/1 -> pot_en_out/1
  Reinterpret1/1 -> Mult/1
  Reinterpret/1 -> Mult/2
  Slice/1 -> Reinterpret/1
  Slice1/1 -> coeff_out/1
  coeff/1 -> Slice1/1, Slice/1
  sync_delay/1 -> sync_out/1
  sync/1 -> sync_delay/1
  Mult/1 -> taps_out/1

== system rfsoc4x2_ospfb_128/pfb_fir_real9/pol1_in1_tap33 ==
  din : Inport
  sync : Inport  Port=2
  coeff : Inport  Port=3
  addr_in : Inport  Port=4
  pot_en_in : Inport  Port=5
  Constant59 : xbsIndex_r4/Constant  const=0  gui_display_data_type=Fixed-point  arith_type=Unsigned  n_bits=16  bin_pt=0  preci_type=Single  exp_width=8  frac_width=24  explicit_period=off  period=1  equ=P=C  opselect=C  inp2=PCIN>>17  opr=+  inp1=P  carry=CIN  dbl_ovrd=off  block_type=constant
  Constant60 : xbsIndex_r4/Constant  const=0  gui_display_data_type=Boolean  arith_type=Boolean  n_bits=144  bin_pt=0  preci_type=Single  exp_width=8  frac_width=24  explicit_period=off  period=1  equ=P=C  opselect=C  inp2=PCIN>>17  opr=+  inp1=P  carry=CIN  dbl_ovrd=off  block_type=constant
  Delay : xbsIndex_r4/Delay  rst=off  infoeditControl=Selection of Reset will increase slice count due to use of real FFs and instead of SRLs  en=off  latency=1  reg_retiming=off  dbl_ovrd=off  block_type=delay
  Delay1 : xbsIndex_r4/Delay  rst=off  infoeditControl=Selection of Reset will increase slice count due to use of real FFs and instead of SRLs  en=off  latency=1  reg_retiming=off  dbl_ovrd=off  block_type=delay
  Dual Port RAM13 : xbsIndex_r4/Dual Port RAM  depth=(2^8) / (2^4)  initVector=0  distributed_mem=Block RAM  init_a=0  init_b=0  rst_a=off  rst_b=off  en_a=off  en_b=off  latency=1  write_mode_A=Read After Write  write_mode_B=Read Before Write  optimize=Area  dbl_ovrd=off  simulation_type=fast_sim  block_type=dpram
  Mult : xbsIndex_r4/Mult  precision=Full  arith_type="Signed  (2's comp)"  n_bits=8  bin_pt=2  quantization=Truncate  overflow=Wrap  en=off  latency=0  use_behavioral_HDL=on  opt=Speed  use_embedded=off  optimum_pipeline=off  pipeline=on  dbl_ovrd=off  use_rpm=on  placement_style=Rectangular shape  block_type=mult
      settings: xl_area=[0, 0, 0, 0, 0, 0, 0]  block_version=9.1.01
  Reinterpret : xbsIndex_r4/Reinterpret  force_arith_type=on  arith_type="Signed  (2's comp)"  force_bin_pt=on  bin_pt=coeff_frac_width  block_type=reinterpret
      settings: infoedit="Changes signal type without altering the binary representation.   You can changed the signal between signed and unsigned, and relocate the binary point.<P><P>Hardware notes: In hardware this block costs nothing.<P><P>Example:  Suppose the input is 6 bits wide, signed, with 2 fractional bits, and the output is forced to unsigned with 0 fractional bits.  Then an input of -2.0 (1110.00 in binary 2's complement) becomes an output of 56 (111000 in binary)."  block_version=9.1.01
  Reinterpret1 : xbsIndex_r4/Reinterpret  force_arith_type=on  arith_type="Signed  (2's comp)"  force_bin_pt=on  bin_pt=data_width - 1  block_type=reinterpret
      settings: infoedit="Changes signal type without altering the binary representation.   You can changed the signal between signed and unsigned, and relocate the binary point.<P><P>Hardware notes: In hardware this block costs nothing.<P><P>Example:  Suppose the input is 6 bits wide, signed, with 2 fractional bits, and the output is forced to unsigned with 0 fractional bits.  Then an input of -2.0 (1110.00 in binary 2's complement) becomes an output of 56 (111000 in binary)."  block_version=9.1.01
  Slice : xbsIndex_r4/Slice  nbits=coeff_width  boolean_output=off  mode=Lower Bit Location + Width  bit1=0  base1=MSB of Input  bit0=0  base0=LSB of Input  dbl_ovrd=off  block_type=slice
      settings: infoedit="Extracts a given range of bits from each input sample and presents it at the output.  The output type is ordinarily unsigned with binary point at zero, but can be Boolean when the slice is one bit wide.<P><P>Hardware notes: In hardware this block costs nothing."  block_version=9.1.01
  Slice1 : xbsIndex_r4/Slice  nbits=0  boolean_output=off  mode=Two Bit Locations  bit1=0  base1=MSB of Input  bit0=coeff_width  base0=LSB of Input  dbl_ovrd=off  block_type=slice
      settings: infoedit="Extracts a given range of bits from each input sample and presents it at the output.  The output type is ordinarily unsigned with binary point at zero, but can be Boolean when the slice is one bit wide.<P><P>Hardware notes: In hardware this block costs nothing."  block_version=9.1.01
  Terminator13 : Terminator
  delay_bram : Subsystem  Commented=on  AncestorBlock=casper_library_delays/delay_bram  mask(delay_bram){DelayLen=delay, bram_latency=bram_latency, use_dsp48=off, async=off}
      mask prompts: DelayLen "Delay By:"; bram_latency "BRAM Latency"; use_dsp48 "Use DSP48"; async "asynchronous operation"
      mask help: A delay block that uses BRAM for its storage.
      mask init:
      | delay_bram_init(gcb, ...
      |     'DelayLen', DelayLen, ...
      |     'bram_latency', bram_latency, ...
      |     'use_dsp48', use_dsp48, ...
      |     'async', async);
      mask Help: eval('xlWeb(''http://casper.berkeley.edu/wiki/Delay_bram'')')
  sync_delay : casper_library_delays/sync_delay  DelayLen=delay
      settings: SourceProductName=CASPER DSP Blockset
  dout : Outport  VectorParamsAs1DForOutWhenUnconnected=off
  sync_out : Outport  Port=2  VectorParamsAs1DForOutWhenUnconnected=off
  coeff_out : Outport  Port=3  VectorParamsAs1DForOutWhenUnconnected=off
  taps_out : Outport  Port=4  VectorParamsAs1DForOutWhenUnconnected=off
  add_out : Outport  Port=5  VectorParamsAs1DForOutWhenUnconnected=off
  pot_en_out : Outport  Port=6  VectorParamsAs1DForOutWhenUnconnected=off
  wires:
  addr_in/1 -> Dual Port RAM13/4, Dual Port RAM13/1, Delay/1
  pot_en_in/1 -> Delay1/1, Dual Port RAM13/3
  Constant59/1 -> Dual Port RAM13/5
  Constant60/1 -> Dual Port RAM13/6
  Dual Port RAM13/1 -> Terminator13/1
  din/1 -> Dual Port RAM13/2, Reinterpret1/1
  Delay/1 -> add_out/1
  Dual Port RAM13/2 -> dout/1
  Delay1/1 -> pot_en_out/1
  Reinterpret1/1 -> Mult/1
  Reinterpret/1 -> Mult/2
  Slice/1 -> Reinterpret/1
  Slice1/1 -> coeff_out/1
  coeff/1 -> Slice1/1, Slice/1
  sync_delay/1 -> sync_out/1
  sync/1 -> sync_delay/1
  Mult/1 -> taps_out/1
